simulink model "site_grid_behavior_ev_charging_v3"  (R2025b)
settings: Solver=ode3  StartTime=0.0  StopTime=86400  FixedStep=300  RelTol=1e-3
Description:
  | Site-level EV charging behavior - ILLUSTRATIVE LAYER.
  | Version 3.0.0 | built 2026-07-27T19:08:03Z | scenario SYN001_2026_baseline | capacity_basis placeholder.
  | All quantitative results come from the MATLAB pipeline (runScenario), not from this model.
settings Model: Creator=runner  LastModifiedBy=runner

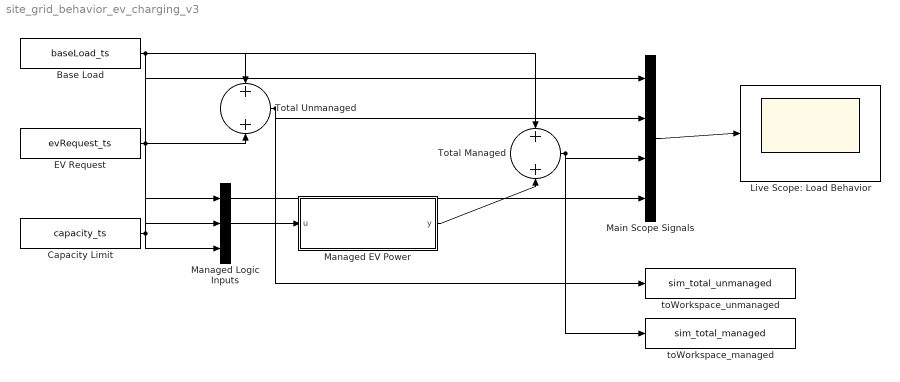
== system site_grid_behavior_ev_charging_v3 ==
  Base Load : FromWorkspace  VariableName=baseLoad_ts
  Capacity Limit : FromWorkspace  VariableName=capacity_ts
  EV Request : FromWorkspace  VariableName=evRequest_ts
  Live Scope: Load Behavior : Scope
  Main Scope Signals : Mux
  Managed EV Power : MATLAB Function  TreatAsAtomicUnit=on
  Managed Logic Inputs : Mux  Inputs=3
  Total Managed : Sum
  Total Unmanaged : Sum
  toWorkspace_managed : ToWorkspace  VariableName=sim_total_managed  SaveFormat=Structure With Time  SampleTime=-1
  toWorkspace_unmanaged : ToWorkspace  VariableName=sim_total_unmanaged  SaveFormat=Structure With Time  SampleTime=-1
  wires:
  Base Load/1 -> Total Unmanaged/1, Managed Logic Inputs/3, Total Managed/1, Main Scope Signals/1
  EV Request/1 -> Total Unmanaged/2, Managed Logic Inputs/1
  Capacity Limit/1 -> Managed Logic Inputs/2, Main Scope Signals/4
  Managed Logic Inputs/1 -> Managed EV Power/1(u)
  Managed EV Power/1(y) -> Total Managed/2
  Total Unmanaged/1 -> Main Scope Signals/2, toWorkspace_unmanaged/1
  Total Managed/1 -> Main Scope Signals/3, toWorkspace_managed/1
  Main Scope Signals/1 -> Live Scope: Load Behavior/1

== matlab function site_grid_behavior_ev_charging_v3/Managed EV Power ==
  data: u input; y output
function y = fcn(u)
% u(1) = EV request, u(2) = capacity, u(3) = base load
% Illustrative clamp only - see managedCharging.m for the
% authoritative strategies incl. the energy-aware scheduler.
available = max(u(2) - u(3), 0);
y = min(u(1), available);
end
